simulink model "PurePursuitControlledRobot"  (R2026a)
settings: Solver=ode1  StopTime=30  FixedStep=2e-5
values from neighbouring files (symbols this model uses):
  goal_v1 = waypoints_v1(end,:).'    [run_simulation.m]
  goal_v2 = waypoints_v2(end,:).'    [run_simulation.m]
  goal_v3 = waypoints_v3(end,:).'    [run_simulation.m]
  tol = 1e-6    (= 1e-06)    [route_planner.m]    (also in run_simulation.m = 0.1)
  waypoints_v1 = W{1}    [run_simulation.m]
  waypoints_v2 = W{2}    [run_simulation.m]
  waypoints_v3 = W{3}    [run_simulation.m]
settings Model: Creator=AdrianStark  LastModifiedBy=AdrianStark

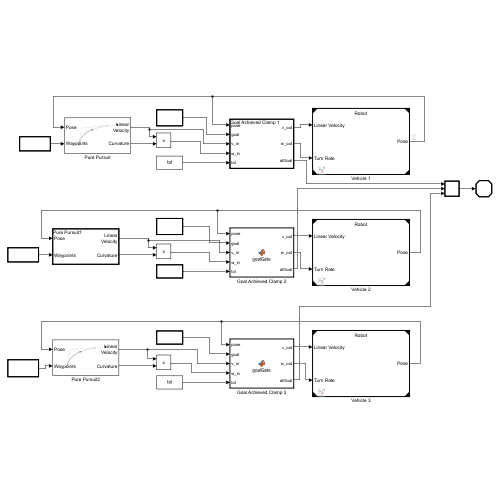
[thumbnail: Simulink's stored preview of the top-level diagram]
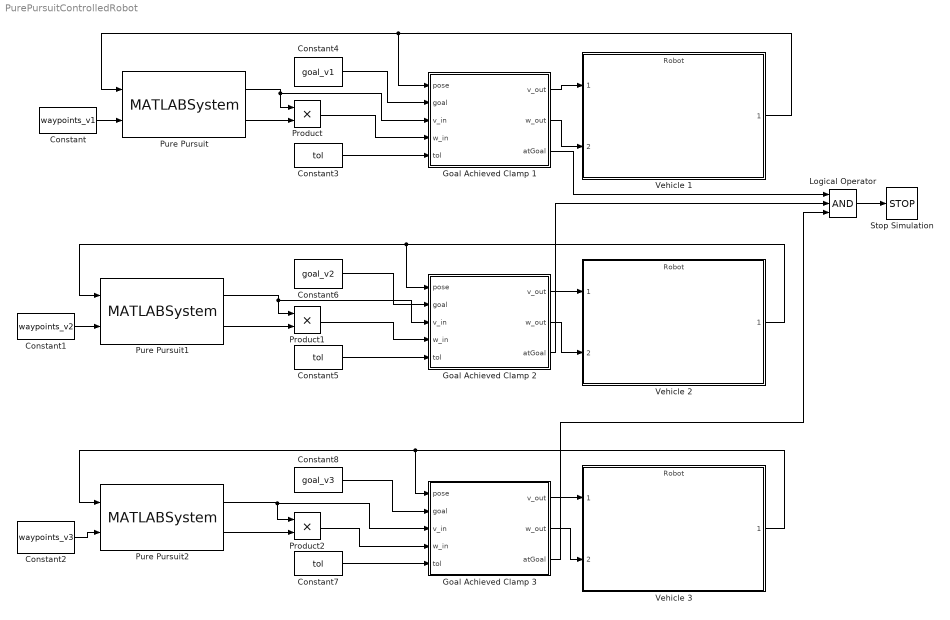
== system PurePursuitControlledRobot ==
  Constant : Constant  Value=waypoints_v1
  Constant1 : Constant  Value=waypoints_v2
  Constant2 : Constant  Value=waypoints_v3
  Constant3 : Constant  Value=tol
  Constant4 : Constant  Value=goal_v1
  Constant5 : Constant  Value=tol
  Constant6 : Constant  Value=goal_v2
  Constant7 : Constant  Value=tol
  Constant8 : Constant  Value=goal_v3
  Goal Achieved Clamp 1 : MATLAB Function  TreatAsAtomicUnit=on
  Goal Achieved Clamp 2 : MATLAB Function  TreatAsAtomicUnit=on
  Goal Achieved Clamp 3 : MATLAB Function  TreatAsAtomicUnit=on
  Logical Operator : Logic  Inputs=3  AllPortsSameDT=off  OutDataTypeStr=boolean
  Product : Product
  Product1 : Product
  Product2 : Product
  Pure Pursuit : MATLABSystem  System=PurePursuitFromStart  DesiredLinearVelocityPort=off  DesiredLinearVelocity=v_desired  MaxCurvature=max_curve  LookaheadDistancePort=off  LookaheadDistance=lookahead  TargetDirPort=off  SimulateUsing=Code generation
      mask Type: PurePursuitFromStart
  Pure Pursuit1 : MATLABSystem  System=PurePursuitFromStart  DesiredLinearVelocityPort=off  DesiredLinearVelocity=v_desired  MaxCurvature=max_curve  LookaheadDistancePort=off  LookaheadDistance=lookahead  TargetDirPort=off  SimulateUsing=Code generation
      mask Type: PurePursuitFromStart
  Pure Pursuit2 : MATLABSystem  System=PurePursuitFromStart  DesiredLinearVelocityPort=off  DesiredLinearVelocity=v_desired  MaxCurvature=max_curve  LookaheadDistancePort=off  LookaheadDistance=lookahead  TargetDirPort=off  SimulateUsing=Code generation
      mask Type: PurePursuitFromStart
  Stop Simulation : Stop
  Vehicle 1 : ModelReference  ModelNameDialog=Robot  UsingDefaultArgumentValue=0,0,0,0,0  ModelReferenceVersion=1.34
  Vehicle 2 : ModelReference  ModelNameDialog=Robot  UsingDefaultArgumentValue=0,0,0,0,0  ModelReferenceVersion=1.34
  Vehicle 3 : ModelReference  ModelNameDialog=Robot  UsingDefaultArgumentValue=0,0,0,0,0  ModelReferenceVersion=1.34
  wires:
  Pure Pursuit/1 -> Goal Achieved Clamp 1/3(v_in), Product/1
  Pure Pursuit1/1 -> Goal Achieved Clamp 2/3(v_in), Product1/1
  Pure Pursuit2/1 -> Goal Achieved Clamp 3/3(v_in), Product2/1
  Constant/1 -> Pure Pursuit/2
  Constant1/1 -> Pure Pursuit1/2
  Constant2/1 -> Pure Pursuit2/2
  Pure Pursuit/2 -> Product/2
  Pure Pursuit2/2 -> Product2/2
  Pure Pursuit1/2 -> Product1/2
  Vehicle 3/1 -> Goal Achieved Clamp 3/1(pose), Pure Pursuit2/1
  Vehicle 2/1 -> Goal Achieved Clamp 2/1(pose), Pure Pursuit1/1
  Product/1 -> Goal Achieved Clamp 1/4(w_in)
  Constant3/1 -> Goal Achieved Clamp 1/5(tol)
  Constant4/1 -> Goal Achieved Clamp 1/2(goal)
  Goal Achieved Clamp 1/1(v_out) -> Vehicle 1/1
  Goal Achieved Clamp 1/2(w_out) -> Vehicle 1/2
  Product1/1 -> Goal Achieved Clamp 2/4(w_in)
  Constant5/1 -> Goal Achieved Clamp 2/5(tol)
  Constant6/1 -> Goal Achieved Clamp 2/2(goal)
  Goal Achieved Clamp 2/1(v_out) -> Vehicle 2/1
  Goal Achieved Clamp 2/2(w_out) -> Vehicle 2/2
  Goal Achieved Clamp 3/2(w_out) -> Vehicle 3/2
  Goal Achieved Clamp 3/1(v_out) -> Vehicle 3/1
  Product2/1 -> Goal Achieved Clamp 3/4(w_in)
  Constant7/1 -> Goal Achieved Clamp 3/5(tol)
  Constant8/1 -> Goal Achieved Clamp 3/2(goal)
  Logical Operator/1 -> Stop Simulation/1
  Goal Achieved Clamp 1/3(atGoal) -> Logical Operator/1
  Goal Achieved Clamp 2/3(atGoal) -> Logical Operator/2
  Goal Achieved Clamp 3/3(atGoal) -> Logical Operator/3
  Vehicle 1/1 -> Goal Achieved Clamp 1/1(pose), Pure Pursuit/1

== matlab function PurePursuitControlledRobot/Goal Achieved Clamp 2 ==
  data: pose input; v_out output; goal input; v_in input; w_in input; tol input; w_out output; atGoal output
function [v_out, w_out, atGoal] = goalGate(pose, goal, v_in, w_in, tol)
% pose : 3x1 [x; y; theta] from the Vehicle
% goal : 2x1 [x; y]  - the last waypoint
% tol  : goal radius [m]

d = hypot(goal(1) - pose(1), goal(2) - pose(2));

if d <= tol
    v_out  = 0;
    w_out  = 0;
    atGoal = 1;
else
    v_out  = v_in;
    w_out  = w_in;
    atGoal = 0;
end
end

== matlab function PurePursuitControlledRobot/Goal Achieved Clamp 1 ==
  data: pose input; v_out output; goal input; v_in input; w_in input; tol input; w_out output; atGoal output
function [v_out, w_out, atGoal] = goalGate(pose, goal, v_in, w_in, tol)
% pose : 3x1 [x; y; theta] from the Vehicle
% goal : 2x1 [x; y]  - the last waypoint
% tol  : goal radius [m]

d = hypot(goal(1) - pose(1), goal(2) - pose(2));

if d <= tol
    v_out  = 0;
    w_out  = 0;
    atGoal = 1;
else
    v_out  = v_in;
    w_out  = w_in;
    atGoal = 0;
end
end

== matlab function PurePursuitControlledRobot/Goal Achieved Clamp 3 ==
  data: pose input; v_out output; goal input; v_in input; w_in input; tol input; w_out output; atGoal output
function [v_out, w_out, atGoal] = goalGate(pose, goal, v_in, w_in, tol)
% pose : 3x1 [x; y; theta] from the Vehicle
% goal : 2x1 [x; y]  - the last waypoint
% tol  : goal radius [m]

d = hypot(goal(1) - pose(1), goal(2) - pose(2));

if d <= tol
    v_out  = 0;
    w_out  = 0;
    atGoal = 1;
else
    v_out  = v_in;
    w_out  = w_in;
    atGoal = 0;
end
end
